simulink model "filtereSensor"  (R2026b)
settings: Solver=FixedStepDiscrete  StopTime=inf  FixedStep=0.1  EnableMultiTasking=on
model workspace (MAT data in the model file):
  PAR_FltUs_Alpha_f32 = Simulink.Parameter
  PAR_FltUs_Alpha_f32.Value = 0.20000000298
  PAR_FltUs_Alpha_f32.Complexity = 'real'
  PAR_FltUs_Alpha_f32.Dimensions = [1 1]
  PAR_FltUs_Alpha_f32.DataType = 'single'
  PAR_FltUs_SigmaBeschl_f32 = Simulink.Parameter
  PAR_FltUs_SigmaBeschl_f32.Value = 0.999710977077
  PAR_FltUs_SigmaBeschl_f32.Complexity = 'real'
  PAR_FltUs_SigmaBeschl_f32.Dimensions = [1 1]
  PAR_FltUs_SigmaBeschl_f32.DataType = 'single'
  PAR_FltUs_SigmaMess_f32 = Simulink.Parameter
  PAR_FltUs_SigmaMess_f32.Value = 0.00288999988697
  PAR_FltUs_SigmaMess_f32.Complexity = 'real'
  PAR_FltUs_SigmaMess_f32.Dimensions = [1 1]
  PAR_FltUs_SigmaMess_f32.DataType = 'single'
  PAR_FltUs_VarGeschw0_f32 = Simulink.Parameter
  PAR_FltUs_VarGeschw0_f32.Value = 100
  PAR_FltUs_VarGeschw0_f32.Complexity = 'real'
  PAR_FltUs_VarGeschw0_f32.Dimensions = [1 1]
  PAR_FltUs_VarGeschw0_f32.DataType = 'single'
  PAR_SenUs_Abtast_f64 = Simulink.Parameter
  PAR_SenUs_Abtast_f64.Value = 0.1
  PAR_SenUs_Abtast_f64.Complexity = 'real'
  PAR_SenUs_Abtast_f64.Dimensions = [1 1]
  PAR_SenUs_Abtast_f64.DataType = 'double'
libraries: arduinosensorlib x1
settings Model: SILPILModeSetting=veronly
settings SolverCC: AutoInsertRateTranBlk=on
settings OptimizationCC: DifferentSizesBufferReuse=on  EfficientTunableParamExpr=on  EnhancedBackFolding=on  MaxStackSize=64  OptimizationCustomize=off  OptimizeBlockOrder=speed  PassReuseOutputArgsAs=Individual arguments  RemoveInternalMemoryZeroInit=on  RemoveRootLevelIOMemoryZeroInit=on
settings DebuggingCC: ParameterTunabilityLossMsg=error
settings HardwareCC: ProdHWDeviceType=Atmel->AVR  ProdLargestAtomicFloat=None
settings SFSimCC: MATLABDynamicMemAlloc=off
settings RTWCC: BuildConfiguration=Faster Runs  Description=Embedded Coder  HardwareBoard=Arduino Uno  SystemTargetFile=ert.tlc  TLCOptions=-aInlineSetEventsForThisBaseRateFcn=TLC_FALSE -aSuppressMultiTaskScheduler=TLC_FALSE -aRateBasedStepFcn=1  TemplateMakefile=ert_default_tmf  Toolchain=Arduino AVR
settings CodeAppCC: ForceParamTrailComments=on  IgnoreCustomStorageClasses=off  InsertBlockDesc=on  OperatorAnnotations=on  SFDataObjDesc=on  SimulinkDataObjDesc=on
settings ERTTargetCC: CombineSignalStateStructs=on  ExtModeAutomaticAllocSize=off  ExtModeIntrfLevel=Level2 - Open  ExtModeMexFile=ext_xcp  ExtModeStaticAlloc=on  SupportContinuousTime=on  SupportVariableSizeSignals=on

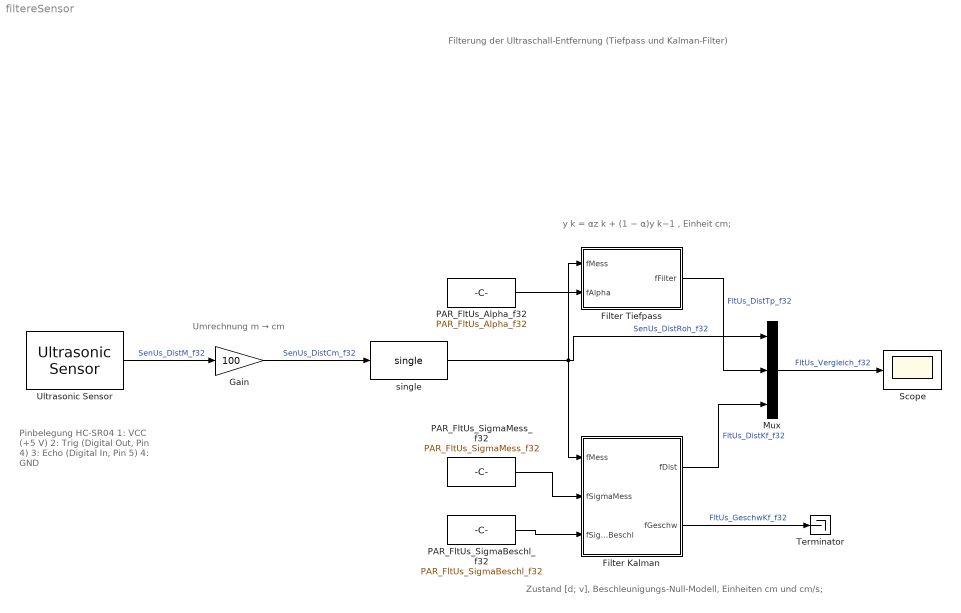
== system filtereSensor ==
  note: Zustand [d; v], Beschleunigungs-Null-Modell, Einheiten cm und cm/s;
  note: y k = αz k + (1 − α)y k−1 , Einheit cm;
  note: Umrechnung m → cm
  note: Pinbelegung HC-SR04
      | 1: VCC (+5 V)
      | 2: Trig (Digital Out, Pin 4)
      | 3: Echo (Digital In, Pin 5)
      | 4: GND
  note: Filterung der Ultraschall-Entfernung (Tiefpass und Kalman-Filter)
  Filter Kalman : MATLAB Function  TreatAsAtomicUnit=on
  Filter Tiefpass : MATLAB Function  TreatAsAtomicUnit=on
  Gain : Gain  Gain=100
  Mux : Mux  Inputs=3
  PAR_FltUs_Alpha_f32 : Constant  Value=PAR_FltUs_Alpha_f32  OutDataTypeStr=single
  PAR_FltUs_SigmaBeschl_f32 : Constant  Value=PAR_FltUs_SigmaBeschl_f32  OutDataTypeStr=single
  PAR_FltUs_SigmaMess_f32 : Constant  Value=PAR_FltUs_SigmaMess_f32  OutDataTypeStr=single
  Scope : Scope
      settings: ActiveDisplayYMinimum=19.593531028437042  ActiveDisplayYMaximum=20.511562515807306
  Terminator : Terminator
  Ultrasonic Sensor : arduinosensorlib/Ultrasonic Sensor  NumSignalPins=2  TrigPin=4  EchoPin=5  SignalPin=3  SampleTime_=PAR_SenUs_Abtast_f64  blockPlatform=ARDUINO
  single : DataTypeConversion  OutDataTypeStr=single  SaturateOnIntegerOverflow=off  RndMeth=Floor
  wires:
  Ultrasonic Sensor/1 -> Gain/1  "SenUs_DistM_f32"
  Gain/1 -> single/1  "SenUs_DistCm_f32"
  single/1 -> Filter Kalman/1(fMess), Filter Tiefpass/1(fMess), Mux/1  "SenUs_DistRoh_f32"
  PAR_FltUs_Alpha_f32/1 -> Filter Tiefpass/2(fAlpha)
  PAR_FltUs_SigmaMess_f32/1 -> Filter Kalman/2(fSigmaMess)
  PAR_FltUs_SigmaBeschl_f32/1 -> Filter Kalman/3(fSigmaBeschl)
  Filter Tiefpass/1(fFilter) -> Mux/2  "FltUs_DistTp_f32"
  Filter Kalman/1(fDist) -> Mux/3  "FltUs_DistKf_f32"
  Filter Kalman/2(fGeschw) -> Terminator/1  "FltUs_GeschwKf_f32"
  Mux/1 -> Scope/1  "FltUs_Vergleich_f32"

== matlab function filtereSensor/Filter Kalman ==
  data: fMess input; fDist output; fSigmaMess input; fSigmaBeschl input; fGeschw output; PAR_SenUs_Abtast_f64 parameter; PAR_FltUs_VarGeschw0_f32 parameter
function [fDist, fGeschw] = fcn(fMess, fSigmaMess, fSigmaBeschl,PAR_SenUs_Abtast_f64, PAR_FltUs_VarGeschw0_f32)
% Kalman-Filter, Beschleunigungs-Null-Modell, x = [d; v]
% Eingang fMess: Entfernung [cm]; 0 = kein Echo
% Eingang fSigmaMess: Messrauschen sigma_z [cm]
% Eingang fSigmaBeschl: Modellrauschen sigma_a [cm/s^2]
% Ausgang fDist: geschaetzte Entfernung [cm]
% Ausgang fGeschw: geschaetzte Geschwindigkeit [cm/s]
persistent afX aP bStart
TS_ABTAST = single(PAR_SenUs_Abtast_f64);    % Abtastzeit [s], muss zum Modell passen
VAR_GESCHW_START = PAR_FltUs_VarGeschw0_f32;   % Startvarianz Geschwindigkeit [cm^2/s^2]

if isempty(bStart)
    bStart = false;
    afX = zeros(2, 1, 'single');
    aP = zeros(2, 2, 'single');
end

aF = single([1, TS_ABTAST; 0, 1]);
aH = single([1, 0]);
aQ = fSigmaBeschl^2 * single([TS_ABTAST^4/4, TS_ABTAST^3/2; ...
                              TS_ABTAST^3/2, TS_ABTAST^2]);
fR = fSigmaMess^2;                 % Messrauschvarianz [cm^2]
bGueltig = fMess > single(0);

if ~bStart
    if bGueltig
        afX = [fMess; single(0)];
        aP = diag([fR, VAR_GESCHW_START]);
        bStart = true;
    end
else
    afX = aF * afX;                % Vorhersage
    aP = aF * aP * aF' + aQ;

    if bGueltig                    % Korrektur nur bei gueltigem Echo
        fS = aH * aP * aH' + fR;
        aK = aP * aH' / fS;
        afX = afX + aK * (fMess - aH * afX);
        aIKH = eye(2, 'single') - aK * aH;
        aP = aIKH * aP * aIKH' + aK * fR * aK';   % Joseph-Form
    end
end
fDist = afX(1);
fGeschw = afX(2);
end

== matlab function filtereSensor/Filter Tiefpass ==
  data: fMess input; fFilter output; fAlpha input
function fFilter = TiefPassUS(fMess, fAlpha)
% Eingang fMess [cm]; 0 = kein Echo zurueck
% Eingang fAlpha: Gewicht des neuen Messwerts
% Ausgang fFilter [cm]: gefilterte Entfernung

persistent fAlt bStart
if isempty(bStart)
    bStart = false;
    fAlt = single(0);
end

if fMess > single(0)
    if ~bStart
        fAlt = fMess;     % Start mit erstem gueltigen Messwert
        bStart = true;
    else
        % y(k) = alpha * z(k) + (1 - alpha) * y(k-1)
        fAlt = fAlpha * fMess + (single(1) - fAlpha) * fAlt;
    end
end
fFilter = fAlt;           % Bei Nullwert bleibt der letzte Wert erhalten
end
